simulink model "KUKA_Dynamics_internal_massonly"  (R2021b)
settings: Solver=ode4  StartTime=0.0  StopTime=0.01  FixedStep=0.01  RelTol=1e-3
InitFcn:
  | % ************** Initiate forces
  | % f0=[0;0;0;0;0;0];
  | % f0=[0;0;0;0;0;0;0];
  | %f_0=[0;0;0];
  | %f_m=[0;0];
  | %f_e=[0;0;0;0;0;0];
  | % ************** Initiate states
  | %q_m=[0;0];
  | %q_dot_m=[0;0];
  | %P=[0;0;0];
  | %V_I0=[0;0;0];
  | % ************** Load main
  | %run(Main.m)
values from neighbouring files (symbols this model uses):
  diag_M = diagonalize(M_frak0, M_frak)    [Create_Robot.m]    (also in Main.m; Main__iiwa7.m; diagonalize.m = zeros(6*(n+1),6*(n+1)); test_C_Main.m)
  f_e = [0;0;0;0;0;0]    [Create_Robot.m]    (also in Main.m = [0;0;0]; Main__iiwa7.m; test_C_Main.m)
  f_m = [0;0]    [Create_Robot.m]    (also in Main.m; Main__iiwa7.m; test_C_Main.m)
  q_dot_m = [0;0]    [Create_Robot.m]    (also in Main.m; Main__iiwa7.m; test_C_Main.m)
  q_m = [0;0]    [Create_Robot.m]    (also in Main.m = [0.2;0.4]; Main__iiwa7.m = [0.2;0.4]; test_C_Main.m = [1;0])
  X = [0 -x(3) x(2) ; x(3) 0 -x(1) ; -x(2) x(1) 0 ]    [skewsym.m]
  Xi_m_matrix = zeros(6*n,n)    [Create_Robot.m]    (also in Main.m; Main__iiwa7.m; test_C_Main.m)
undefined symbols (not defined in the file or in its folder): Xi_m, Y, Z
libraries: sm_lib x78, nesl_utility x29
(part 1 of 2)
settings Model: Creator=Bmmog  LastModifiedBy=Bmmog
settings SolverCC: AllowMultiTaskInputOutput=on

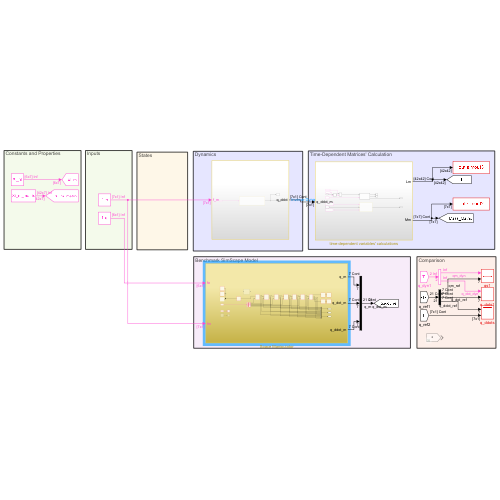
[thumbnail: Simulink's stored preview of the top-level diagram]
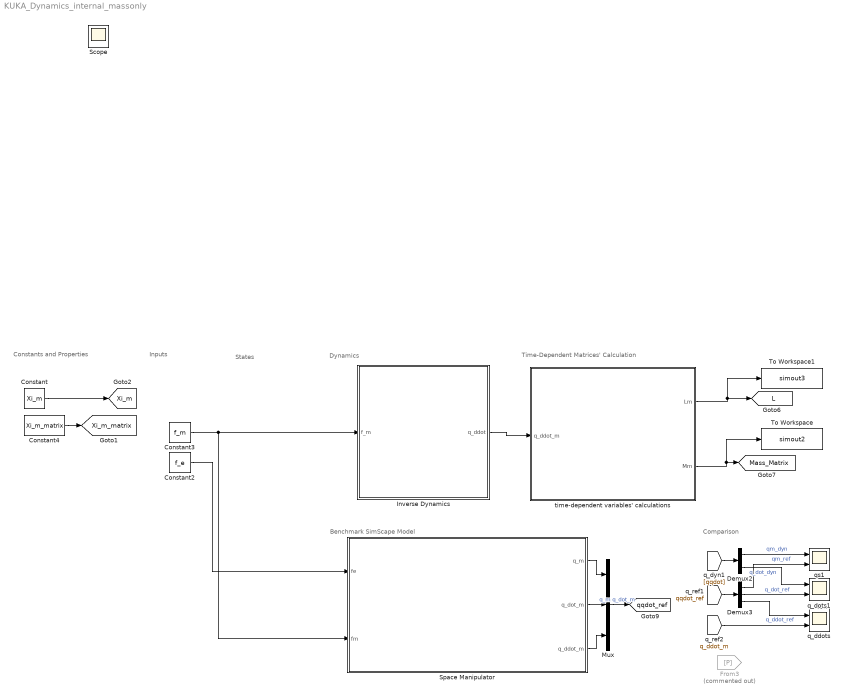
== system KUKA_Dynamics_internal_massonly ==
  note: Time-Dependent Matrices' Calculation
  note: States
  note: Inputs
  note: Dynamics
  note: Constants and Properties
  note: Benchmark SimScape Model
  note: Comparison
  Constant : Constant  Value=Xi_m  VectorParams1D=off
  Constant2 : Constant  Value=f_e  VectorParams1D=off
  Constant3 : Constant  Value=f_m  VectorParams1D=off
  Constant4 : Constant  Value=Xi_m_matrix  VectorParams1D=off
  Demux2 : Demux  Outputs=2
  Demux3 : Demux  Outputs=3
  From3 : From  Commented=on  GotoTag=P  TagVisibility=global
  Inverse Dynamics : Subsystem
  Mux : Mux  Inputs=3
  Space Manipulator : Subsystem
  To Workspace : ToWorkspace  VariableName=simout2  SaveFormat=Timeseries  SampleTime=-1
  To Workspace1 : ToWorkspace  VariableName=simout3  SaveFormat=Timeseries  SampleTime=-1
  q_ddots : Scope  NumInputPorts=2
  q_dots1 : Scope  NumInputPorts=2
  qs1 : Scope  NumInputPorts=2
  time-dependent variables' calculations : Subsystem
  Scope : Scope
  tag scope: L=global, Mass_Matrix=global, Xi_m=global, Xi_m_matrix=global, qqdot_ref=global
  wires:
  Constant/1 -> [Xi_m]
  Constant4/1 -> [Xi_m_matrix]
  time-dependent variables' calculations/2(Mm) -> To Workspace/1, [Mass_Matrix]
  time-dependent variables' calculations/1(Lm) -> To Workspace1/1, [L]
  Inverse Dynamics/1(q_ddot) -> time-dependent variables' calculations/1(q_ddot_m)
  Mux/1 -> [qqdot_ref]  "q_m q_dot_m"
  Constant2/1 -> Space Manipulator/1(fe)
  Space Manipulator/1(q_m) -> Mux/1
  Space Manipulator/2(q_dot_m) -> Mux/2
  Constant3/1 -> Space Manipulator/2(fm), Inverse Dynamics/1(f_m)
  Demux3/2 -> q_dots1/2  "q_dot_ref"
  [qqdot] -> Demux2/1
  Demux3/1 -> qs1/2  "qm_ref"
  Demux2/2 -> q_dots1/1  "q_dot_dyn"
  [qqdot_ref] -> Demux3/1
  Demux2/1 -> qs1/1  "qm_dyn"
  Space Manipulator/3(q_ddot_m) -> Mux/3
  Demux3/3 -> q_ddots/1  "q_ddot_ref"
  [q_ddot_m] -> q_ddots/2

== system KUKA_Dynamics_internal_massonly/Inverse Dynamics ==
  f_m : Inport
  Internal Dynamics : Subsystem
  q_ddot : Outport
  tag scope: q_ddot_m=global
  wires:
  f_m/1 -> Internal Dynamics/1(f_m)
  Internal Dynamics/1(q_ddot) -> [q_ddot_m], q_ddot/1  "q_ddot"

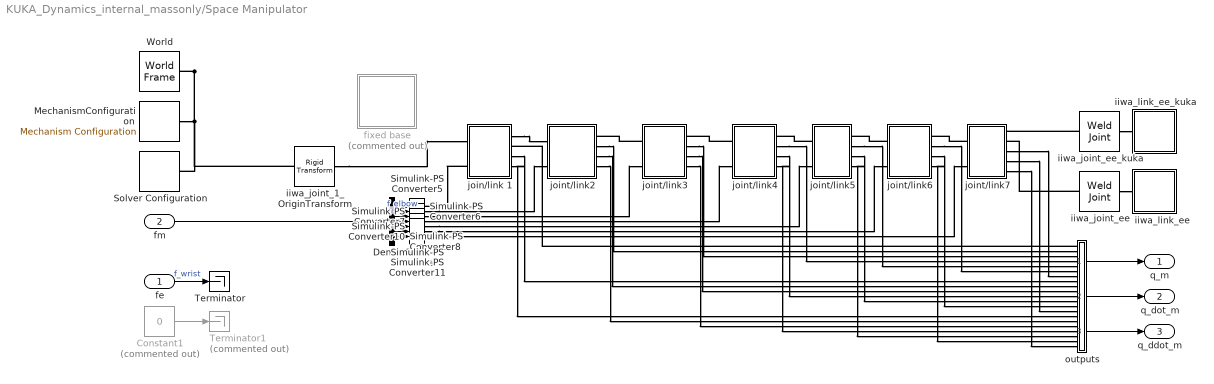
== system KUKA_Dynamics_internal_massonly/Space Manipulator ==
  fe : Inport
  fm : Inport  Port=2
  Constant1 : Constant  Commented=on  Value=0
  Demux2 : Demux  Outputs=7
  MechanismConfiguration : sm_lib/Utilities/Mechanism Configuration  UniformGravity=Constant  GravityVector=[0 0 0]  GravityUnits=m/s^2  LinearizationDelta=0.001  JointModeTransitionNonlinearIterations=2
  Simulink-PS Converter{5..11} (7 alike) : nesl_utility/Simulink-PS Converter  PhysicalDomain=network_engine_domain  SubClassName=ps_input  LeftPortType=input  RightPortType=output  PseudoPeriodic=off  Frequencies=[]  NoiseDistribution=none  NoiseParameters=[]  Unit=1  AffineConversion=off  FilteringAndDerivatives=provide  SimscapeFilterOrder=1  InputFilterTimeConstant=0.001  UdotUserProvided=0
      settings: SourceProductBaseCode=PW,SS
  Solver Configuration : nesl_utility/Solver Configuration  PhysicalDomain=network_engine_domain  SubClassName=solver  LeftPortType=input  RightPortType=generic  Tones=[]  Harmonics=[]  SimulateNoise=off  Profile=off  UseLocalSampling=off  EnableSwitchedLinearOptims=on  FrequencyDomain=off  UseCCode=off  RelTol=0.001  AbsTol=0.001  MinStep=1e-09  ToWorkspace=off  RevertToSquareIcSolve=off  NumHomotopyIterations=100  PhasorMode=off  PhasorModeNumHarmonics=1  DoDC=off  ResidualTolerance=1e-09  UseLocalSolver=off  LocalSolverChoice=NE_BACKWARD_EULER_ADVANCER  LocalSolverSampleTime=0.001  DoFixedCost=off  MaxNonlinIter=3  MaxModeIter=2  ComputeImpulses=off  ImpulseIterations=2  LinearAlgebra=auto  EquationFormulation=NE_TIME_EF  DelaysMemoryBudget=1024  AutomaticFiltering=on  FilteringTimeConstant=0.001  PartitionStorageMethod=AS_NEEDED  PartitionMemoryBudget=1024  PartitionMethod=ROBUST
      settings: SourceProductBaseCode=PW,SS
  Terminator : Terminator
  Terminator1 : Terminator  Commented=on
  World : sm_lib/Frames and Transforms/World Frame
  fixed base : Subsystem  Commented=on
  iiwa_joint_1_OriginTransform : sm_lib/Frames and Transforms/Rigid Transform  TranslationMethod=Cartesian  TranslationStandardOffset=0  TranslationLengthUnit=m  TranslationStandardAxis=+Z  TranslationCartesianOffset=[0, 0, 0]  TranslationROffset=0  TranslationROffsetUnits=m  TranslationZOffset=0  TranslationZOffsetUnits=m  TranslationThetaOffset=0  TranslationThetaOffsetUnits=deg  RotationMethod=RotationSequence  RotationAngleUnits=deg  RotationStandardAxis=+Z  RotationAngle=0.0  RotationArbitraryAxis=[0 0 1]  FollAlignAxisA=+X  BaseAlignAxisA=+Y  FollAlignAxisB=+Y  BaseAlignAxisB=+Z  RotationSequenceAxes=BaseAxes  RotationSequence=XYZ  RotationSequenceAngles=[0, 0, 0]  RotationSequenceAnglesUnits=rad  RotationMatrix=[1 0 0; 0 1 0; 0 0 1]
  iiwa_joint_ee : sm_lib/Joints/Weld Joint  JointMode=Normal  SenseConstraintForce=off  SenseConstraintForceX=off  SenseConstraintForceY=off  SenseConstraintForceZ=off  SenseConstraintTorque=off  SenseConstraintTorqueX=off  SenseConstraintTorqueY=off  SenseConstraintTorqueZ=off  SenseTotalForce=off  SenseTotalForceX=off  SenseTotalForceY=off  SenseTotalForceZ=off  SenseTotalTorque=off  SenseTotalTorqueX=off  SenseTotalTorqueY=off  SenseTotalTorqueZ=off  CompositeWrenchDir=FollowerOnBase  CompositeWrenchFrame=BaseFrame
  iiwa_joint_ee_kuka : sm_lib/Joints/Weld Joint  JointMode=Normal  SenseConstraintForce=off  SenseConstraintForceX=off  SenseConstraintForceY=off  SenseConstraintForceZ=off  SenseConstraintTorque=off  SenseConstraintTorqueX=off  SenseConstraintTorqueY=off  SenseConstraintTorqueZ=off  SenseTotalForce=off  SenseTotalForceX=off  SenseTotalForceY=off  SenseTotalForceZ=off  SenseTotalTorque=off  SenseTotalTorqueX=off  SenseTotalTorqueY=off  SenseTotalTorqueZ=off  CompositeWrenchDir=FollowerOnBase  CompositeWrenchFrame=BaseFrame
  iiwa_link_ee : Subsystem
  iiwa_link_ee_kuka : Subsystem
  join/link 1 : Subsystem
  joint/link2 : Subsystem
  joint/link3 : Subsystem
  joint/link4 : Subsystem
  joint/link5 : Subsystem
  joint/link6 : Subsystem
  joint/link7 : Subsystem
  outputs : Subsystem
  q_m : Outport
  q_dot_m : Outport  Port=2
  q_ddot_m : Outport  Port=3
  wires:
  fe/1 -> Terminator/1  "f_wrist"
  Demux2/7 -> Simulink-PS Converter11/1
  Demux2/1 -> Simulink-PS Converter5/1
  Demux2/5 -> Simulink-PS Converter9/1
  Demux2/2 -> Simulink-PS Converter6/1  "f_elbow"
  Constant1/1 -> Terminator1/1
  Demux2/4 -> Simulink-PS Converter8/1
  Demux2/6 -> Simulink-PS Converter10/1
  Demux2/3 -> Simulink-PS Converter7/1
  fm/1 -> Demux2/1
  outputs/1(q_m) -> q_m/1
  outputs/2(q_dot_m) -> q_dot_m/1
  outputs/3(q_ddot_m) -> q_ddot_m/1
  connections:
  World/RConn1 -- iiwa_joint_1_OriginTransform/LConn1 -- Solver Configuration/RConn1 -- MechanismConfiguration/RConn1
  joint/link7/RConn5 -- outputs/LConn21
  Simulink-PS Converter9/RConn1 -- joint/link5/LConn2
  Simulink-PS Converter7/RConn1 -- joint/link3/LConn2
  joint/link7/RConn4 -- outputs/LConn14
  joint/link3/RConn3 -- outputs/LConn10
  joint/link4/LConn1 -- joint/link3/RConn1
  join/link 1/RConn1 -- joint/link2/LConn1
  joint/link5/RConn4 -- outputs/LConn19
  outputs/LConn1 -- join/link 1/RConn2
  joint/link5/RConn2 -- outputs/LConn5
  joint/link6/RConn2 -- outputs/LConn6
  joint/link5/RConn3 -- outputs/LConn12
  joint/link7/LConn1 -- joint/link6/RConn1
  iiwa_joint_ee_kuka/LConn1 -- joint/link7/RConn1
  iiwa_joint_ee/RConn1 -- iiwa_link_ee/LConn1
  joint/link2/RConn2 -- outputs/LConn2
  joint/link2/RConn4 -- outputs/LConn16
  iiwa_joint_ee_kuka/RConn1 -- iiwa_link_ee_kuka/LConn1
  Simulink-PS Converter6/RConn1 -- joint/link2/LConn2
  joint/link4/RConn4 -- outputs/LConn18
  joint/link7/RConn3 -- outputs/LConn7
  Simulink-PS Converter8/RConn1 -- joint/link4/LConn2
  joint/link3/LConn1 -- joint/link2/RConn1
  iiwa_joint_ee/LConn1 -- joint/link7/RConn2
  join/link 1/RConn4 -- outputs/LConn15
  Simulink-PS Converter10/RConn1 -- joint/link6/LConn2
  joint/link3/RConn2 -- outputs/LConn3
  joint/link3/RConn4 -- outputs/LConn17
  joint/link6/RConn4 -- outputs/LConn20
  joint/link4/RConn2 -- outputs/LConn4
  joint/link6/LConn1 -- joint/link5/RConn1
  joint/link5/LConn1 -- joint/link4/RConn1
  join/link 1/RConn3 -- outputs/LConn8
  joint/link2/RConn3 -- outputs/LConn9
  joint/link6/RConn3 -- outputs/LConn13
  joint/link4/RConn3 -- outputs/LConn11
  Simulink-PS Converter11/RConn1 -- joint/link7/LConn2
  iiwa_joint_1_OriginTransform/RConn1 -- join/link 1/LConn1
  join/link 1/LConn2 -- Simulink-PS Converter5/RConn1

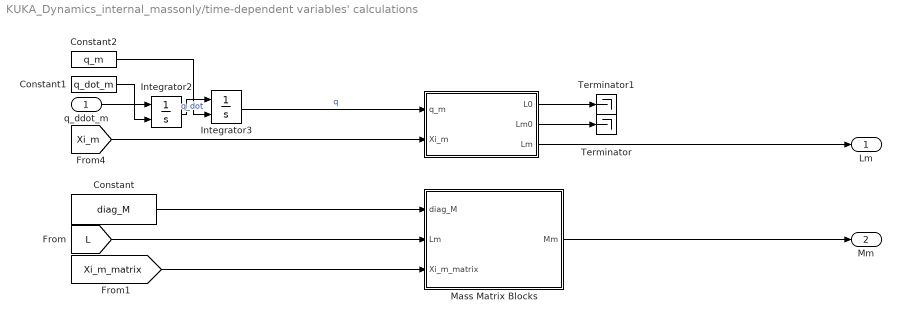
== system KUKA_Dynamics_internal_massonly/time-dependent variables' calculations ==
  q_ddot_m : Inport
  " " : MATLAB Function  TreatAsAtomicUnit=on
  Constant : Constant  Value=diag_M  VectorParams1D=off
  Constant1 : Constant  Value=q_dot_m  VectorParams1D=off
  Constant2 : Constant  Value=q_m  VectorParams1D=off
  Integrator2 : Integrator  InitialConditionSource=external  InitialCondition=q_dot_m
  Integrator3 : Integrator  InitialConditionSource=external
  Mass Matrix Blocks : Subsystem
  Terminator : Terminator
  Terminator1 : Terminator
  Lm : Outport
  Mm : Outport  Port=2
  wires:
  Mass Matrix Blocks/1(Mm) -> Mm/1
  Integrator2/1 -> Integrator3/1  "q_dot"
  q_ddot_m/1 -> Integrator2/1
  " "/1(L0) -> Terminator1/1
  " "/3(Lm) -> Lm/1
  " "/2(Lm0) -> Terminator/1
  Constant/1 -> Mass Matrix Blocks/1(diag_M)
  [L] -> Mass Matrix Blocks/2(Lm)
  [Xi_m_matrix] -> Mass Matrix Blocks/3(Xi_m_matrix)
  [Xi_m] -> " "/2(Xi_m)
  Integrator3/1 -> " "/1(q_m)  "q"
  Constant1/1 -> Integrator2/2
  Constant2/1 -> Integrator3/2

== system KUKA_Dynamics_internal_massonly/Inverse Dynamics/Internal Dynamics ==
  f_m : Inport
  Divide : Product  Inputs=/*  Multiplication=Matrix(*)
  To Workspace : ToWorkspace  VariableName=qddot  SaveFormat=Timeseries  SampleTime=-1
  q_ddot : Outport
  wires:
  f_m/1 -> Divide/2
  Divide/1 -> To Workspace/1, q_ddot/1
  [Mass_Matrix] -> Divide/1

== system KUKA_Dynamics_internal_massonly/Space Manipulator/fixed base ==
  iiwa_link_0 : Subsystem
  world_iiwa_joint : sm_lib/Joints/Weld Joint  JointMode=Normal  SenseConstraintForce=off  SenseConstraintForceX=off  SenseConstraintForceY=off  SenseConstraintForceZ=off  SenseConstraintTorque=off  SenseConstraintTorqueX=off  SenseConstraintTorqueY=off  SenseConstraintTorqueZ=off  SenseTotalForce=off  SenseTotalForceX=off  SenseTotalForceY=off  SenseTotalForceZ=off  SenseTotalTorque=off  SenseTotalTorqueX=off  SenseTotalTorqueY=off  SenseTotalTorqueZ=off  CompositeWrenchDir=FollowerOnBase  CompositeWrenchFrame=BaseFrame
  F1 : PMIOPort  Side=Right
  Conn2 : PMIOPort  Port=2  Side=Left
  connections:
  iiwa_link_0/LConn1 -- world_iiwa_joint/RConn1
  Conn2/RConn1 -- world_iiwa_joint/LConn1
  F1/RConn1 -- iiwa_link_0/RConn1

== system KUKA_Dynamics_internal_massonly/Space Manipulator/iiwa_link_ee ==
  ReferenceFrame : sm_lib/Frames and Transforms/Reference Frame
  F : PMIOPort  Side=Left
  connections:
  ReferenceFrame/RConn1 -- F/RConn1

== system KUKA_Dynamics_internal_massonly/Space Manipulator/iiwa_link_ee_kuka ==
  ReferenceFrame : sm_lib/Frames and Transforms/Reference Frame
  F : PMIOPort  Side=Left
  connections:
  ReferenceFrame/RConn1 -- F/RConn1

== system KUKA_Dynamics_internal_massonly/Space Manipulator/join//link 1 ==
  iiwa_joint_1 : sm_lib/Joints/Revolute Joint  JointMode=Normal  SenseConstraintForce=off  SenseConstraintForceX=off  SenseConstraintForceY=off  SenseConstraintForceZ=off  SenseConstraintTorque=off  SenseConstraintTorqueX=off  SenseConstraintTorqueY=off  SenseConstraintTorqueZ=off  SenseTotalForce=off  SenseTotalForceX=off  SenseTotalForceY=off  SenseTotalForceZ=off  SenseTotalTorque=off  SenseTotalTorqueX=off  SenseTotalTorqueY=off  SenseTotalTorqueZ=off  CompositeWrenchDir=FollowerOnBase  CompositeWrenchFrame=BaseFrame  EquilibriumPosition=0  EquilibriumPositionUnits=deg  SpringStiffness=0  SpringStiffnessUnits=N*m/deg  DampingCoefficient=0.5  DampingCoefficientUnits=kg*m^2/(rad*s)  TorqueActuationMode=InputTorque  MotionActuationMode=ComputedMotion  SensePosition=on  SenseVelocity=on  SenseAcceleration=on  SenseTorqueForce=off  SenseLowerLimitTorqueForce=off  SenseUpperLimitTorqueForce=off  LowerLimitSpecify=on  LowerLimitBound=-2.96705972839  LowerLimitBoundUnits=rad  LowerLimitStiffness=1e4  LowerLimitStiffnessUnits=N*m/deg  LowerLimitDamping=10  LowerLimitDampingUnits=N*m/(deg/s)  LowerLimitTransitionRegionWidth=0.1  LowerLimitTransitionRegionWidthUnits=deg  UpperLimitSpecify=on  UpperLimitBound=2.96705972839  UpperLimitBoundUnits=rad  UpperLimitStiffness=1e4  UpperLimitStiffnessUnits=N*m/deg  UpperLimitDamping=10  UpperLimitDampingUnits=N*m/(deg/s)  UpperLimitTransitionRegionWidth=0.1  UpperLimitTransitionRegionWidthUnits=deg  PositionTargetSpecify=on  PositionTargetPriority=High  PositionTargetValue=q_m(1)  PositionTargetValueUnits=rad  VelocityTargetSpecify=on  VelocityTargetPriority=High  VelocityTargetValue=0  VelocityTargetValueUnits=rad/s
  iiwa_link_1 : Subsystem
  b : PMIOPort  Side=Left
  f1 : PMIOPort  Port=2  Side=Left
  F1 : PMIOPort  Port=3  Side=Right
  q1 : PMIOPort  Port=4  Side=Right
  qd1 : PMIOPort  Port=5  Side=Right
  qdd1 : PMIOPort  Port=6  Side=Right
  connections:
  iiwa_joint_1/RConn1 -- iiwa_link_1/LConn1
  iiwa_joint_1/LConn1 -- b/RConn1
  iiwa_joint_1/RConn2 -- q1/RConn1
  f1/RConn1 -- iiwa_joint_1/LConn2
  iiwa_joint_1/RConn3 -- qd1/RConn1
  iiwa_joint_1/RConn4 -- qdd1/RConn1
  F1/RConn1 -- iiwa_link_1/RConn1

== system KUKA_Dynamics_internal_massonly/Space Manipulator/joint//link2 ==
  iiwa_joint_2 : sm_lib/Joints/Revolute Joint  JointMode=Normal  SenseConstraintForce=off  SenseConstraintForceX=off  SenseConstraintForceY=off  SenseConstraintForceZ=off  SenseConstraintTorque=off  SenseConstraintTorqueX=off  SenseConstraintTorqueY=off  SenseConstraintTorqueZ=off  SenseTotalForce=off  SenseTotalForceX=off  SenseTotalForceY=off  SenseTotalForceZ=off  SenseTotalTorque=off  SenseTotalTorqueX=off  SenseTotalTorqueY=off  SenseTotalTorqueZ=off  CompositeWrenchDir=FollowerOnBase  CompositeWrenchFrame=BaseFrame  EquilibriumPosition=0  EquilibriumPositionUnits=deg  SpringStiffness=0  SpringStiffnessUnits=N*m/deg  DampingCoefficient=0.5  DampingCoefficientUnits=kg*m^2/(rad*s)  TorqueActuationMode=InputTorque  MotionActuationMode=ComputedMotion  SensePosition=on  SenseVelocity=on  SenseAcceleration=on  SenseTorqueForce=off  SenseLowerLimitTorqueForce=off  SenseUpperLimitTorqueForce=off  LowerLimitSpecify=on  LowerLimitBound=-2.09439510239  LowerLimitBoundUnits=rad  LowerLimitStiffness=1e4  LowerLimitStiffnessUnits=N*m/deg  LowerLimitDamping=10  LowerLimitDampingUnits=N*m/(deg/s)  LowerLimitTransitionRegionWidth=0.1  LowerLimitTransitionRegionWidthUnits=deg  UpperLimitSpecify=on  UpperLimitBound=2.09439510239  UpperLimitBoundUnits=rad  UpperLimitStiffness=1e4  UpperLimitStiffnessUnits=N*m/deg  UpperLimitDamping=10  UpperLimitDampingUnits=N*m/(deg/s)  UpperLimitTransitionRegionWidth=0.1  UpperLimitTransitionRegionWidthUnits=deg  PositionTargetSpecify=on  PositionTargetPriority=High  PositionTargetValue=q_m(2)  PositionTargetValueUnits=rad  VelocityTargetSpecify=on  VelocityTargetPriority=High  VelocityTargetValue=0  VelocityTargetValueUnits=rad/s
  iiwa_link_2 : Subsystem
  b : PMIOPort  Side=Left
  F1 : PMIOPort  Port=2  Side=Right
  f2 : PMIOPort  Port=3  Side=Left
  q2 : PMIOPort  Port=4  Side=Right
  qd2 : PMIOPort  Port=5  Side=Right
  qdd2 : PMIOPort  Port=6  Side=Right
  connections:
  iiwa_joint_2/RConn3 -- qd2/RConn1
  iiwa_joint_2/RConn1 -- iiwa_link_2/LConn1
  F1/RConn1 -- iiwa_link_2/RConn1
  iiwa_joint_2/RConn4 -- qdd2/RConn1
  iiwa_joint_2/LConn1 -- b/RConn1
  f2/RConn1 -- iiwa_joint_2/LConn2
  iiwa_joint_2/RConn2 -- q2/RConn1

== system KUKA_Dynamics_internal_massonly/Space Manipulator/joint//link3 ==
  iiwa_joint_3 : sm_lib/Joints/Revolute Joint  JointMode=Normal  SenseConstraintForce=off  SenseConstraintForceX=off  SenseConstraintForceY=off  SenseConstraintForceZ=off  SenseConstraintTorque=off  SenseConstraintTorqueX=off  SenseConstraintTorqueY=off  SenseConstraintTorqueZ=off  SenseTotalForce=off  SenseTotalForceX=off  SenseTotalForceY=off  SenseTotalForceZ=off  SenseTotalTorque=off  SenseTotalTorqueX=off  SenseTotalTorqueY=off  SenseTotalTorqueZ=off  CompositeWrenchDir=FollowerOnBase  CompositeWrenchFrame=BaseFrame  EquilibriumPosition=0  EquilibriumPositionUnits=deg  SpringStiffness=0  SpringStiffnessUnits=N*m/deg  DampingCoefficient=0.5  DampingCoefficientUnits=kg*m^2/(rad*s)  TorqueActuationMode=InputTorque  MotionActuationMode=ComputedMotion  SensePosition=on  SenseVelocity=on  SenseAcceleration=on  SenseTorqueForce=off  SenseLowerLimitTorqueForce=off  SenseUpperLimitTorqueForce=off  LowerLimitSpecify=on  LowerLimitBound=-2.96705972839  LowerLimitBoundUnits=rad  LowerLimitStiffness=1e4  LowerLimitStiffnessUnits=N*m/deg  LowerLimitDamping=10  LowerLimitDampingUnits=N*m/(deg/s)  LowerLimitTransitionRegionWidth=0.1  LowerLimitTransitionRegionWidthUnits=deg  UpperLimitSpecify=on  UpperLimitBound=2.96705972839  UpperLimitBoundUnits=rad  UpperLimitStiffness=1e4  UpperLimitStiffnessUnits=N*m/deg  UpperLimitDamping=10  UpperLimitDampingUnits=N*m/(deg/s)  UpperLimitTransitionRegionWidth=0.1  UpperLimitTransitionRegionWidthUnits=deg  PositionTargetSpecify=on  PositionTargetPriority=High  PositionTargetValue=q_m(3)  PositionTargetValueUnits=rad  VelocityTargetSpecify=on  VelocityTargetPriority=High  VelocityTargetValue=0  VelocityTargetValueUnits=rad/s
  iiwa_link_3 : Subsystem
  b : PMIOPort  Side=Left
  F1 : PMIOPort  Port=2  Side=Right
  f3 : PMIOPort  Port=3  Side=Left
  q3 : PMIOPort  Port=4  Side=Right
  qd3 : PMIOPort  Port=5  Side=Right
  qdd3 : PMIOPort  Port=6  Side=Right
  connections:
  iiwa_joint_3/RConn1 -- iiwa_link_3/LConn1
  iiwa_joint_3/RConn4 -- qdd3/RConn1
  iiwa_joint_3/RConn3 -- qd3/RConn1
  iiwa_joint_3/RConn2 -- q3/RConn1
  F1/RConn1 -- iiwa_link_3/RConn1
  f3/RConn1 -- iiwa_joint_3/LConn2
  iiwa_joint_3/LConn1 -- b/RConn1

== system KUKA_Dynamics_internal_massonly/Space Manipulator/joint//link4 ==
  iiwa_joint_4 : sm_lib/Joints/Revolute Joint  JointMode=Normal  SenseConstraintForce=off  SenseConstraintForceX=off  SenseConstraintForceY=off  SenseConstraintForceZ=off  SenseConstraintTorque=off  SenseConstraintTorqueX=off  SenseConstraintTorqueY=off  SenseConstraintTorqueZ=off  SenseTotalForce=off  SenseTotalForceX=off  SenseTotalForceY=off  SenseTotalForceZ=off  SenseTotalTorque=off  SenseTotalTorqueX=off  SenseTotalTorqueY=off  SenseTotalTorqueZ=off  CompositeWrenchDir=FollowerOnBase  CompositeWrenchFrame=BaseFrame  EquilibriumPosition=0  EquilibriumPositionUnits=deg  SpringStiffness=0  SpringStiffnessUnits=N*m/deg  DampingCoefficient=0.5  DampingCoefficientUnits=kg*m^2/(rad*s)  TorqueActuationMode=InputTorque  MotionActuationMode=ComputedMotion  SensePosition=on  SenseVelocity=on  SenseAcceleration=on  SenseTorqueForce=off  SenseLowerLimitTorqueForce=off  SenseUpperLimitTorqueForce=off  LowerLimitSpecify=on  LowerLimitBound=-2.09439510239  LowerLimitBoundUnits=rad  LowerLimitStiffness=1e4  LowerLimitStiffnessUnits=N*m/deg  LowerLimitDamping=10  LowerLimitDampingUnits=N*m/(deg/s)  LowerLimitTransitionRegionWidth=0.1  LowerLimitTransitionRegionWidthUnits=deg  UpperLimitSpecify=on  UpperLimitBound=2.09439510239  UpperLimitBoundUnits=rad  UpperLimitStiffness=1e4  UpperLimitStiffnessUnits=N*m/deg  UpperLimitDamping=10  UpperLimitDampingUnits=N*m/(deg/s)  UpperLimitTransitionRegionWidth=0.1  UpperLimitTransitionRegionWidthUnits=deg  PositionTargetSpecify=on  PositionTargetPriority=High  PositionTargetValue=q_m(4)  PositionTargetValueUnits=rad  VelocityTargetSpecify=on  VelocityTargetPriority=High  VelocityTargetValue=0  VelocityTargetValueUnits=rad/s
  iiwa_link_4 : Subsystem
  b : PMIOPort  Side=Left
  F1 : PMIOPort  Port=2  Side=Right
  f4 : PMIOPort  Port=3  Side=Left
  q4 : PMIOPort  Port=4  Side=Right
  qd4 : PMIOPort  Port=5  Side=Right
  qd5 : PMIOPort  Port=6  Side=Right
  connections:
  iiwa_joint_4/RConn1 -- iiwa_link_4/LConn1
  iiwa_joint_4/RConn3 -- qd4/RConn1
  f4/RConn1 -- iiwa_joint_4/LConn2
  F1/RConn1 -- iiwa_link_4/RConn1
  iiwa_joint_4/RConn2 -- q4/RConn1
  iiwa_joint_4/LConn1 -- b/RConn1
  iiwa_joint_4/RConn4 -- qd5/RConn1

== system KUKA_Dynamics_internal_massonly/Space Manipulator/joint//link5 ==
  iiwa_joint_5 : sm_lib/Joints/Revolute Joint  JointMode=Normal  SenseConstraintForce=off  SenseConstraintForceX=off  SenseConstraintForceY=off  SenseConstraintForceZ=off  SenseConstraintTorque=off  SenseConstraintTorqueX=off  SenseConstraintTorqueY=off  SenseConstraintTorqueZ=off  SenseTotalForce=off  SenseTotalForceX=off  SenseTotalForceY=off  SenseTotalForceZ=off  SenseTotalTorque=off  SenseTotalTorqueX=off  SenseTotalTorqueY=off  SenseTotalTorqueZ=off  CompositeWrenchDir=FollowerOnBase  CompositeWrenchFrame=BaseFrame  EquilibriumPosition=0  EquilibriumPositionUnits=deg  SpringStiffness=0  SpringStiffnessUnits=N*m/deg  DampingCoefficient=0.5  DampingCoefficientUnits=kg*m^2/(rad*s)  TorqueActuationMode=InputTorque  MotionActuationMode=ComputedMotion  SensePosition=on  SenseVelocity=on  SenseAcceleration=on  SenseTorqueForce=off  SenseLowerLimitTorqueForce=off  SenseUpperLimitTorqueForce=off  LowerLimitSpecify=on  LowerLimitBound=-2.96705972839  LowerLimitBoundUnits=rad  LowerLimitStiffness=1e4  LowerLimitStiffnessUnits=N*m/deg  LowerLimitDamping=10  LowerLimitDampingUnits=N*m/(deg/s)  LowerLimitTransitionRegionWidth=0.1  LowerLimitTransitionRegionWidthUnits=deg  UpperLimitSpecify=on  UpperLimitBound=2.96705972839  UpperLimitBoundUnits=rad  UpperLimitStiffness=1e4  UpperLimitStiffnessUnits=N*m/deg  UpperLimitDamping=10  UpperLimitDampingUnits=N*m/(deg/s)  UpperLimitTransitionRegionWidth=0.1  UpperLimitTransitionRegionWidthUnits=deg  PositionTargetSpecify=on  PositionTargetPriority=High  PositionTargetValue=q_m(5)  PositionTargetValueUnits=rad  VelocityTargetSpecify=on  VelocityTargetPriority=High  VelocityTargetValue=0  VelocityTargetValueUnits=rad/s
  iiwa_link_5 : Subsystem
  b : PMIOPort  Side=Left
  F1 : PMIOPort  Port=2  Side=Right
  f5 : PMIOPort  Port=3  Side=Left
  q5 : PMIOPort  Port=4  Side=Right
  qd5 : PMIOPort  Port=5  Side=Right
  qdd5 : PMIOPort  Port=6  Side=Right
  connections:
  iiwa_joint_5/LConn1 -- b/RConn1
  iiwa_joint_5/RConn2 -- q5/RConn1
  iiwa_joint_5/RConn4 -- qdd5/RConn1
  iiwa_joint_5/RConn1 -- iiwa_link_5/LConn1
  iiwa_joint_5/RConn3 -- qd5/RConn1
  f5/RConn1 -- iiwa_joint_5/LConn2
  F1/RConn1 -- iiwa_link_5/RConn1

== system KUKA_Dynamics_internal_massonly/Space Manipulator/joint//link6 ==
  iiwa_joint_6 : sm_lib/Joints/Revolute Joint  JointMode=Normal  SenseConstraintForce=off  SenseConstraintForceX=off  SenseConstraintForceY=off  SenseConstraintForceZ=off  SenseConstraintTorque=off  SenseConstraintTorqueX=off  SenseConstraintTorqueY=off  SenseConstraintTorqueZ=off  SenseTotalForce=off  SenseTotalForceX=off  SenseTotalForceY=off  SenseTotalForceZ=off  SenseTotalTorque=off  SenseTotalTorqueX=off  SenseTotalTorqueY=off  SenseTotalTorqueZ=off  CompositeWrenchDir=FollowerOnBase  CompositeWrenchFrame=BaseFrame  EquilibriumPosition=0  EquilibriumPositionUnits=deg  SpringStiffness=0  SpringStiffnessUnits=N*m/deg  DampingCoefficient=0.5  DampingCoefficientUnits=kg*m^2/(rad*s)  TorqueActuationMode=InputTorque  MotionActuationMode=ComputedMotion  SensePosition=on  SenseVelocity=on  SenseAcceleration=on  SenseTorqueForce=off  SenseLowerLimitTorqueForce=off  SenseUpperLimitTorqueForce=off  LowerLimitSpecify=on  LowerLimitBound=-2.09439510239  LowerLimitBoundUnits=rad  LowerLimitStiffness=1e4  LowerLimitStiffnessUnits=N*m/deg  LowerLimitDamping=10  LowerLimitDampingUnits=N*m/(deg/s)  LowerLimitTransitionRegionWidth=0.1  LowerLimitTransitionRegionWidthUnits=deg  UpperLimitSpecify=on  UpperLimitBound=2.09439510239  UpperLimitBoundUnits=rad  UpperLimitStiffness=1e4  UpperLimitStiffnessUnits=N*m/deg  UpperLimitDamping=10  UpperLimitDampingUnits=N*m/(deg/s)  UpperLimitTransitionRegionWidth=0.1  UpperLimitTransitionRegionWidthUnits=deg  PositionTargetSpecify=on  PositionTargetPriority=High  PositionTargetValue=q_m(6)  PositionTargetValueUnits=rad  VelocityTargetSpecify=on  VelocityTargetPriority=High  VelocityTargetValue=0  VelocityTargetValueUnits=rad/s
  iiwa_link_6 : Subsystem
  b : PMIOPort  Side=Left
  F1 : PMIOPort  Port=2  Side=Right
  q6 : PMIOPort  Port=3  Side=Right
  f6 : PMIOPort  Port=4  Side=Left
  qd6 : PMIOPort  Port=5  Side=Right
  qdd6 : PMIOPort  Port=6  Side=Right
  connections:
  iiwa_joint_6/RConn1 -- iiwa_link_6/LConn1
  iiwa_joint_6/LConn1 -- b/RConn1
  F1/RConn1 -- iiwa_link_6/RConn1
  f6/RConn1 -- iiwa_joint_6/LConn2
  iiwa_joint_6/RConn4 -- qdd6/RConn1
  iiwa_joint_6/RConn3 -- qd6/RConn1
  iiwa_joint_6/RConn2 -- q6/RConn1

== system KUKA_Dynamics_internal_massonly/Space Manipulator/joint//link7 ==
  iiwa_joint_7 : sm_lib/Joints/Revolute Joint  JointMode=Normal  SenseConstraintForce=off  SenseConstraintForceX=off  SenseConstraintForceY=off  SenseConstraintForceZ=off  SenseConstraintTorque=off  SenseConstraintTorqueX=off  SenseConstraintTorqueY=off  SenseConstraintTorqueZ=off  SenseTotalForce=off  SenseTotalForceX=off  SenseTotalForceY=off  SenseTotalForceZ=off  SenseTotalTorque=off  SenseTotalTorqueX=off  SenseTotalTorqueY=off  SenseTotalTorqueZ=off  CompositeWrenchDir=FollowerOnBase  CompositeWrenchFrame=BaseFrame  EquilibriumPosition=0  EquilibriumPositionUnits=deg  SpringStiffness=0  SpringStiffnessUnits=N*m/deg  DampingCoefficient=0.5  DampingCoefficientUnits=kg*m^2/(rad*s)  TorqueActuationMode=InputTorque  MotionActuationMode=ComputedMotion  SensePosition=on  SenseVelocity=on  SenseAcceleration=on  SenseTorqueForce=off  SenseLowerLimitTorqueForce=off  SenseUpperLimitTorqueForce=off  LowerLimitSpecify=on  LowerLimitBound=-3.05432619099  LowerLimitBoundUnits=rad  LowerLimitStiffness=1e4  LowerLimitStiffnessUnits=N*m/deg  LowerLimitDamping=10  LowerLimitDampingUnits=N*m/(deg/s)  LowerLimitTransitionRegionWidth=0.1  LowerLimitTransitionRegionWidthUnits=deg  UpperLimitSpecify=on  UpperLimitBound=3.05432619099  UpperLimitBoundUnits=rad  UpperLimitStiffness=1e4  UpperLimitStiffnessUnits=N*m/deg  UpperLimitDamping=10  UpperLimitDampingUnits=N*m/(deg/s)  UpperLimitTransitionRegionWidth=0.1  UpperLimitTransitionRegionWidthUnits=deg  PositionTargetSpecify=on  PositionTargetPriority=High  PositionTargetValue=q_m(7)  PositionTargetValueUnits=rad  VelocityTargetSpecify=on  VelocityTargetPriority=High  VelocityTargetValue=0  VelocityTargetValueUnits=rad/s
  iiwa_link_7 : Subsystem
  F2 : PMIOPort  Side=Right
  b : PMIOPort  Port=2  Side=Left
  F1 : PMIOPort  Port=3  Side=Right
  q7 : PMIOPort  Port=4  Side=Right
  f7 : PMIOPort  Port=5  Side=Left
  qd7 : PMIOPort  Port=6  Side=Right
  qdd7 : PMIOPort  Port=7  Side=Right
  connections:
  iiwa_joint_7/RConn1 -- iiwa_link_7/LConn1
  iiwa_joint_7/RConn4 -- qdd7/RConn1
  iiwa_joint_7/RConn2 -- q7/RConn1
  iiwa_joint_7/RConn3 -- qd7/RConn1
  f7/RConn1 -- iiwa_joint_7/LConn2
  F1/RConn1 -- iiwa_link_7/RConn2
  F2/RConn1 -- iiwa_link_7/RConn1
  iiwa_joint_7/LConn1 -- b/RConn1

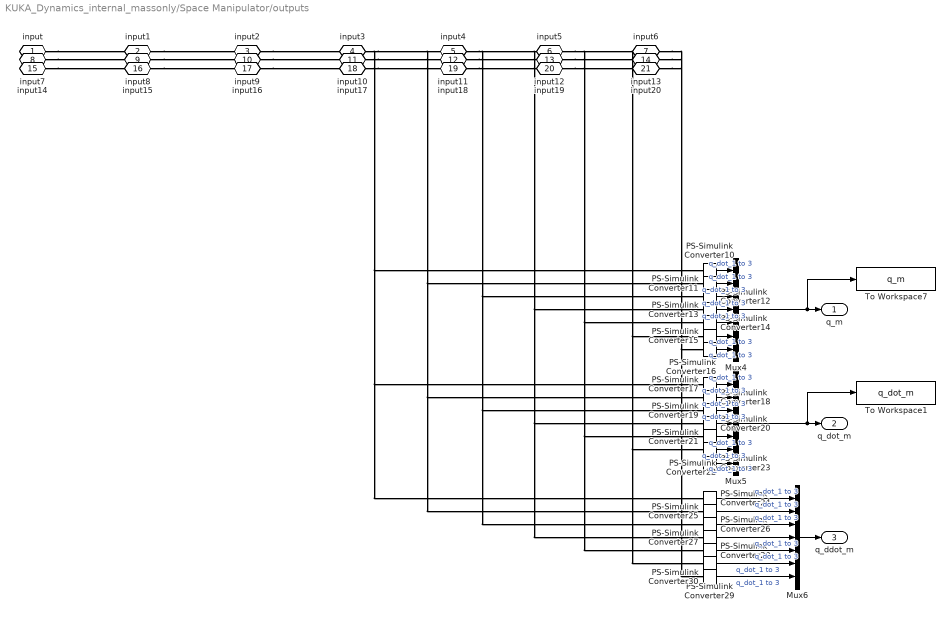
== system KUKA_Dynamics_internal_massonly/Space Manipulator/outputs ==
  Mux4 : Mux  Inputs=7
  Mux5 : Mux  Inputs=7
  Mux6 : Mux  Inputs=7
  PS-Simulink Converter{10..30} (21 alike) : nesl_utility/PS-Simulink Converter  PhysicalDomain=network_engine_domain  SubClassName=ps_output  LeftPortType=input  RightPortType=output  PseudoPeriodic=off  Frequencies=[]  Unit=inherit  AffineConversion=off
      settings: SourceProductBaseCode=PW,SS
  To Workspace1 : ToWorkspace  VariableName=q_dot_m  SampleTime=-1
  To Workspace7 : ToWorkspace  VariableName=q_m  SampleTime=-1
  input : PMIOPort  Side=Left
  input1 : PMIOPort  Port=2  Side=Left
  input2 : PMIOPort  Port=3  Side=Left
  input3 : PMIOPort  Port=4  Side=Left
  input4 : PMIOPort  Port=5  Side=Left
  input5 : PMIOPort  Port=6  Side=Left
  input6 : PMIOPort  Port=7  Side=Left
  input7 : PMIOPort  Port=8  Side=Left
  input8 : PMIOPort  Port=9  Side=Left
  input9 : PMIOPort  Port=10  Side=Left
  input10 : PMIOPort  Port=11  Side=Left
  input11 : PMIOPort  Port=12  Side=Left
  input12 : PMIOPort  Port=13  Side=Left
  input13 : PMIOPort  Port=14  Side=Left
  input14 : PMIOPort  Port=15  Side=Left
  input15 : PMIOPort  Port=16  Side=Left
  input16 : PMIOPort  Port=17  Side=Left
  input17 : PMIOPort  Port=18  Side=Left
  input18 : PMIOPort  Port=19  Side=Left
  input19 : PMIOPort  Port=20  Side=Left
  input20 : PMIOPort  Port=21  Side=Left
  q_m : Outport
  q_dot_m : Outport  Port=2
  q_ddot_m : Outport  Port=3
  wires:
  PS-Simulink Converter21/1 -> Mux5/5  "q_dot_1 to 3"
  PS-Simulink Converter12/1 -> Mux4/3  "q_dot_1 to 3"
  PS-Simulink Converter29/1 -> Mux6/6  "q_dot_1 to 3"
  PS-Simulink Converter14/1 -> Mux4/5  "q_dot_1 to 3"
  PS-Simulink Converter26/1 -> Mux6/3  "q_dot_1 to 3"
  PS-Simulink Converter17/1 -> Mux5/1  "q_dot_1 to 3"
  PS-Simulink Converter11/1 -> Mux4/2  "q_dot_1 to 3"
  PS-Simulink Converter25/1 -> Mux6/2  "q_dot_1 to 3"
  PS-Simulink Converter24/1 -> Mux6/1  "q_dot_1 to 3"
  PS-Simulink Converter10/1 -> Mux4/1  "q_dot_1 to 3"
  PS-Simulink Converter27/1 -> Mux6/4  "q_dot_1 to 3"
  PS-Simulink Converter28/1 -> Mux6/5  "q_dot_1 to 3"
  PS-Simulink Converter15/1 -> Mux4/6  "q_dot_1 to 3"
  PS-Simulink Converter16/1 -> Mux4/7  "q_dot_1 to 3"
  PS-Simulink Converter18/1 -> Mux5/2  "q_dot_1 to 3"
  PS-Simulink Converter30/1 -> Mux6/7  "q_dot_1 to 3"
  PS-Simulink Converter13/1 -> Mux4/4  "q_dot_1 to 3"
  PS-Simulink Converter22/1 -> Mux5/6  "q_dot_1 to 3"
  PS-Simulink Converter23/1 -> Mux5/7  "q_dot_1 to 3"
  PS-Simulink Converter20/1 -> Mux5/4  "q_dot_1 to 3"
  PS-Simulink Converter19/1 -> Mux5/3  "q_dot_1 to 3"
  Mux5/1 -> To Workspace1/1, q_dot_m/1
  Mux6/1 -> q_ddot_m/1
  Mux4/1 -> To Workspace7/1, q_m/1
  connections:
  input7/RConn1 -- PS-Simulink Converter17/LConn1
  input11/RConn1 -- PS-Simulink Converter21/LConn1
  input20/RConn1 -- PS-Simulink Converter30/LConn1
  input16/RConn1 -- PS-Simulink Converter26/LConn1
  input2/RConn1 -- PS-Simulink Converter12/LConn1
  input10/RConn1 -- PS-Simulink Converter20/LConn1
  input17/RConn1 -- PS-Simulink Converter27/LConn1
  input18/RConn1 -- PS-Simulink Converter28/LConn1
  input/RConn1 -- PS-Simulink Converter10/LConn1
  input19/RConn1 -- PS-Simulink Converter29/LConn1
  input5/RConn1 -- PS-Simulink Converter15/LConn1
  input14/RConn1 -- PS-Simulink Converter24/LConn1
  input6/RConn1 -- PS-Simulink Converter16/LConn1
  input9/RConn1 -- PS-Simulink Converter19/LConn1
  input8/RConn1 -- PS-Simulink Converter18/LConn1
  input15/RConn1 -- PS-Simulink Converter25/LConn1
  input12/RConn1 -- PS-Simulink Converter22/LConn1
  input13/RConn1 -- PS-Simulink Converter23/LConn1
  input1/RConn1 -- PS-Simulink Converter11/LConn1
  input4/RConn1 -- PS-Simulink Converter14/LConn1
  input3/RConn1 -- PS-Simulink Converter13/LConn1

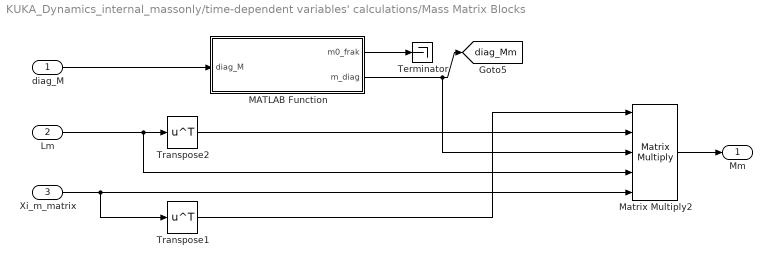
== system KUKA_Dynamics_internal_massonly/time-dependent variables' calculations/Mass Matrix Blocks ==
  diag_M : Inport
  Lm : Inport  Port=2
  Xi_m_matrix : Inport  Port=3
  MATLAB Function : MATLAB Function  TreatAsAtomicUnit=on
  Matrix Multiply2 : Product  Inputs=5  Multiplication=Matrix(*)
  Terminator : Terminator
  Transpose1 : Math  Operator=transpose  SaturateOnIntegerOverflow=on
  Transpose2 : Math  Operator=transpose  SaturateOnIntegerOverflow=on
  Mm : Outport
  tag scope: diag_Mm=global
  wires:
  Matrix Multiply2/1 -> Mm/1
  Xi_m_matrix/1 -> Transpose1/1, Matrix Multiply2/5
  diag_M/1 -> MATLAB Function/1(diag_M)
  Lm/1 -> Matrix Multiply2/4, Transpose2/1
  Transpose1/1 -> Matrix Multiply2/1
  Transpose2/1 -> Matrix Multiply2/2
  MATLAB Function/1(m0_frak) -> Terminator/1
  MATLAB Function/2(m_diag) -> [diag_Mm], Matrix Multiply2/3

== system KUKA_Dynamics_internal_massonly/Space Manipulator/fixed base/iiwa_link_0 ==
  Inertia : sm_lib/Body Elements/Inertia  InertiaType=Custom  Mass=5  MassUnits=kg  CenterOfMass=[0, 0, 0]  CenterOfMassUnits=m  MomentsOfInertia=[0.05, 0.06, 0.03]  MomentsOfInertiaUnits=kg*m^2  ProductsOfInertia=[0, 0, 0]  ProductsOfInertiaUnits=kg*m^2  GraphicType=None  MarkerShape=Inertia  MarkerSize=20  GraphicVisPropType=SimpleVisualProperties  GraphicDiffuseColor=[0.5 0.5 0.5]  GraphicSpecularColor=[0.5 0.5 0.5 1.0]  GraphicAmbientColor=[0.15 0.15 0.15 1.0]  GraphicEmissiveColor=[0.0 0.0 0.0 1.0]  GraphicShininess=75  GraphicOpacity=1.0
  InertiaOriginTransform : sm_lib/Frames and Transforms/Rigid Transform  TranslationMethod=Cartesian  TranslationStandardOffset=0  TranslationLengthUnit=m  TranslationStandardAxis=+Z  TranslationCartesianOffset=[-0.1, 0, 0.07000000000000001]  TranslationROffset=0  TranslationROffsetUnits=m  TranslationZOffset=0  TranslationZOffsetUnits=m  TranslationThetaOffset=0  TranslationThetaOffsetUnits=deg  RotationMethod=RotationSequence  RotationAngleUnits=deg  RotationStandardAxis=+Z  RotationAngle=0.0  RotationArbitraryAxis=[0 0 1]  FollAlignAxisA=+X  BaseAlignAxisA=+Y  FollAlignAxisB=+Y  BaseAlignAxisB=+Z  RotationSequenceAxes=BaseAxes  RotationSequence=XYZ  RotationSequenceAngles=[0, 0, 0]  RotationSequenceAnglesUnits=rad  RotationMatrix=[1 0 0; 0 1 0; 0 0 1]
  ReferenceFrame : sm_lib/Frames and Transforms/Reference Frame
  Visual : sm_lib/Body Elements/File Solid  ExtGeomFileName=iiwa_description/meshes/iiwa7/visual/link_0.stl  UnitType=Custom  ExtGeomFileUnits=m  StepReaderType=HEX  ExportConvexHullGeometry=off  InertiaType=Custom  Mass=0  MassUnits=kg  CenterOfMass=[0, 0, 0]  CenterOfMassUnits=m  MomentsOfInertia=[0, 0, 0]  MomentsOfInertiaUnits=kg*m^2  ProductsOfInertia=[0, 0, 0]  ProductsOfInertiaUnits=kg*m^2  BasedOnType=DensityFromFile  Density=1000  DensityUnits=kg/m^3  DoExposeReferenceFrame=on  SerializedFrames=<Frames/>  GraphicType=FromGeometry  MarkerShape=Sphere  MarkerSize=10  GraphicVisPropType=SimpleVisualProperties  GraphicDiffuseColor=[0.4, 0.4, 0.4]  GraphicSpecularColor=[0.5 0.5 0.5 1.0]  GraphicAmbientColor=[0.15 0.15 0.15 1.0]  GraphicEmissiveColor=[0.0 0.0 0.0 1.0]  GraphicShininess=75  GraphicOpacity=1
  VisualOriginTransform : sm_lib/Frames and Transforms/Rigid Transform  TranslationMethod=Cartesian  TranslationStandardOffset=0  TranslationLengthUnit=m  TranslationStandardAxis=+Z  TranslationCartesianOffset=[0, 0, 0]  TranslationROffset=0  TranslationROffsetUnits=m  TranslationZOffset=0  TranslationZOffsetUnits=m  TranslationThetaOffset=0  TranslationThetaOffsetUnits=deg  RotationMethod=RotationSequence  RotationAngleUnits=deg  RotationStandardAxis=+Z  RotationAngle=0.0  RotationArbitraryAxis=[0 0 1]  FollAlignAxisA=+X  BaseAlignAxisA=+Y  FollAlignAxisB=+Y  BaseAlignAxisB=+Z  RotationSequenceAxes=BaseAxes  RotationSequence=XYZ  RotationSequenceAngles=[0, 0, 0]  RotationSequenceAnglesUnits=rad  RotationMatrix=[1 0 0; 0 1 0; 0 0 1]
  iiwa_joint_1_AxisTransform : sm_lib/Frames and Transforms/Rigid Transform  TranslationMethod=Cartesian  TranslationStandardOffset=0  TranslationLengthUnit=m  TranslationStandardAxis=+Z  TranslationCartesianOffset=[0, 0, 0]  TranslationROffset=0  TranslationROffsetUnits=m  TranslationZOffset=0  TranslationZOffsetUnits=m  TranslationThetaOffset=0  TranslationThetaOffsetUnits=deg  RotationMethod=ArbitraryAxis  RotationAngleUnits=rad  RotationStandardAxis=+Z  RotationAngle=0  RotationArbitraryAxis=[1, 0, 0]  FollAlignAxisA=+X  BaseAlignAxisA=+Y  FollAlignAxisB=+Y  BaseAlignAxisB=+Z  RotationSequenceAxes=FollowerAxes  RotationSequence=XYX  RotationSequenceAngles=[0 0 0]  RotationSequenceAnglesUnits=deg  RotationMatrix=[1 0 0; 0 1 0; 0 0 1]
  iiwa_joint_1_OriginTransform : sm_lib/Frames and Transforms/Rigid Transform  TranslationMethod=Cartesian  TranslationStandardOffset=0  TranslationLengthUnit=m  TranslationStandardAxis=+Z  TranslationCartesianOffset=[0, 0, 0.02]  TranslationROffset=0  TranslationROffsetUnits=m  TranslationZOffset=0  TranslationZOffsetUnits=m  TranslationThetaOffset=0  TranslationThetaOffsetUnits=deg  RotationMethod=RotationSequence  RotationAngleUnits=deg  RotationStandardAxis=+Z  RotationAngle=0.0  RotationArbitraryAxis=[0 0 1]  FollAlignAxisA=+X  BaseAlignAxisA=+Y  FollAlignAxisB=+Y  BaseAlignAxisB=+Z  RotationSequenceAxes=BaseAxes  RotationSequence=XYZ  RotationSequenceAngles=[0, 0, 0]  RotationSequenceAnglesUnits=rad  RotationMatrix=[1 0 0; 0 1 0; 0 0 1]
  F : PMIOPort  Side=Left
  F1 : PMIOPort  Port=2  Side=Right
  connections:
  Inertia/RConn1 -- InertiaOriginTransform/RConn1
  InertiaOriginTransform/LConn1 -- ReferenceFrame/RConn1 -- F/RConn1 -- VisualOriginTransform/LConn1 -- iiwa_joint_1_OriginTransform/LConn1
  Visual/RConn1 -- VisualOriginTransform/RConn1
  iiwa_joint_1_AxisTransform/RConn1 -- F1/RConn1
  iiwa_joint_1_AxisTransform/LConn1 -- iiwa_joint_1_OriginTransform/RConn1

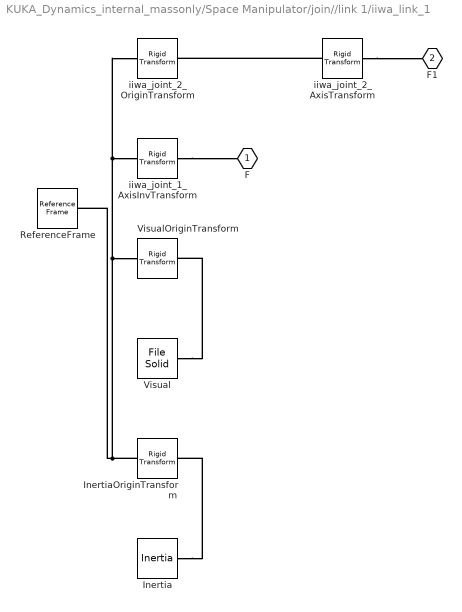
== system KUKA_Dynamics_internal_massonly/Space Manipulator/join//link 1/iiwa_link_1 ==
  Inertia : sm_lib/Body Elements/Inertia  InertiaType=Custom  Mass=3.4525  MassUnits=kg  CenterOfMass=[0, 0, 0]  CenterOfMassUnits=m  MomentsOfInertia=[0.02183, 0.007703, 0.02083]  MomentsOfInertiaUnits=kg*m^2  ProductsOfInertia=[-0.003887, 0, 0]  ProductsOfInertiaUnits=kg*m^2  GraphicType=None  MarkerShape=Inertia  MarkerSize=20  GraphicVisPropType=SimpleVisualProperties  GraphicDiffuseColor=[0.5 0.5 0.5]  GraphicSpecularColor=[0.5 0.5 0.5 1.0]  GraphicAmbientColor=[0.15 0.15 0.15 1.0]  GraphicEmissiveColor=[0.0 0.0 0.0 1.0]  GraphicShininess=75  GraphicOpacity=1.0
  InertiaOriginTransform : sm_lib/Frames and Transforms/Rigid Transform  TranslationMethod=Cartesian  TranslationStandardOffset=0  TranslationLengthUnit=m  TranslationStandardAxis=+Z  TranslationCartesianOffset=[0, -0.03, 0.12]  TranslationROffset=0  TranslationROffsetUnits=m  TranslationZOffset=0  TranslationZOffsetUnits=m  TranslationThetaOffset=0  TranslationThetaOffsetUnits=deg  RotationMethod=RotationSequence  RotationAngleUnits=deg  RotationStandardAxis=+Z  RotationAngle=0.0  RotationArbitraryAxis=[0 0 1]  FollAlignAxisA=+X  BaseAlignAxisA=+Y  FollAlignAxisB=+Y  BaseAlignAxisB=+Z  RotationSequenceAxes=BaseAxes  RotationSequence=XYZ  RotationSequenceAngles=[0, 0, 0]  RotationSequenceAnglesUnits=rad  RotationMatrix=[1 0 0; 0 1 0; 0 0 1]
  ReferenceFrame : sm_lib/Frames and Transforms/Reference Frame
  Visual : sm_lib/Body Elements/File Solid  ExtGeomFileName=iiwa_description/meshes/iiwa7/visual/link_1.stl  UnitType=Custom  ExtGeomFileUnits=m  StepReaderType=HEX  ExportConvexHullGeometry=off  InertiaType=Custom  Mass=0  MassUnits=kg  CenterOfMass=[0, 0, 0]  CenterOfMassUnits=m  MomentsOfInertia=[0, 0, 0]  MomentsOfInertiaUnits=kg*m^2  ProductsOfInertia=[0, 0, 0]  ProductsOfInertiaUnits=kg*m^2  BasedOnType=DensityFromFile  Density=1000  DensityUnits=kg/m^3  DoExposeReferenceFrame=on  SerializedFrames=<Frames/>  GraphicType=FromGeometry  MarkerShape=Sphere  MarkerSize=10  GraphicVisPropType=SimpleVisualProperties  GraphicDiffuseColor=[1, 0.423529411765, 0.0392156862745]  GraphicSpecularColor=[0.5 0.5 0.5 1.0]  GraphicAmbientColor=[0.15 0.15 0.15 1.0]  GraphicEmissiveColor=[0.0 0.0 0.0 1.0]  GraphicShininess=75  GraphicOpacity=1
  VisualOriginTransform : sm_lib/Frames and Transforms/Rigid Transform  TranslationMethod=Cartesian  TranslationStandardOffset=0  TranslationLengthUnit=m  TranslationStandardAxis=+Z  TranslationCartesianOffset=[0, 0, 0]  TranslationROffset=0  TranslationROffsetUnits=m  TranslationZOffset=0  TranslationZOffsetUnits=m  TranslationThetaOffset=0  TranslationThetaOffsetUnits=deg  RotationMethod=RotationSequence  RotationAngleUnits=deg  RotationStandardAxis=+Z  RotationAngle=0.0  RotationArbitraryAxis=[0 0 1]  FollAlignAxisA=+X  BaseAlignAxisA=+Y  FollAlignAxisB=+Y  BaseAlignAxisB=+Z  RotationSequenceAxes=BaseAxes  RotationSequence=XYZ  RotationSequenceAngles=[0, 0, 0]  RotationSequenceAnglesUnits=rad  RotationMatrix=[1 0 0; 0 1 0; 0 0 1]
  iiwa_joint_1_AxisInvTransform : sm_lib/Frames and Transforms/Rigid Transform  TranslationMethod=Cartesian  TranslationStandardOffset=0  TranslationLengthUnit=m  TranslationStandardAxis=+Z  TranslationCartesianOffset=[0, 0, 0]  TranslationROffset=0  TranslationROffsetUnits=m  TranslationZOffset=0  TranslationZOffsetUnits=m  TranslationThetaOffset=0  TranslationThetaOffsetUnits=deg  RotationMethod=ArbitraryAxis  RotationAngleUnits=rad  RotationStandardAxis=+Z  RotationAngle=0  RotationArbitraryAxis=[1, 0, 0]  FollAlignAxisA=+X  BaseAlignAxisA=+Y  FollAlignAxisB=+Y  BaseAlignAxisB=+Z  RotationSequenceAxes=FollowerAxes  RotationSequence=XYX  RotationSequenceAngles=[0 0 0]  RotationSequenceAnglesUnits=deg  RotationMatrix=[1 0 0; 0 1 0; 0 0 1]
  iiwa_joint_2_AxisTransform : sm_lib/Frames and Transforms/Rigid Transform  TranslationMethod=Cartesian  TranslationStandardOffset=0  TranslationLengthUnit=m  TranslationStandardAxis=+Z  TranslationCartesianOffset=[0, 0, 0]  TranslationROffset=0  TranslationROffsetUnits=m  TranslationZOffset=0  TranslationZOffsetUnits=m  TranslationThetaOffset=0  TranslationThetaOffsetUnits=deg  RotationMethod=ArbitraryAxis  RotationAngleUnits=rad  RotationStandardAxis=+Z  RotationAngle=0  RotationArbitraryAxis=[1, 0, 0]  FollAlignAxisA=+X  BaseAlignAxisA=+Y  FollAlignAxisB=+Y  BaseAlignAxisB=+Z  RotationSequenceAxes=FollowerAxes  RotationSequence=XYX  RotationSequenceAngles=[0 0 0]  RotationSequenceAnglesUnits=deg  RotationMatrix=[1 0 0; 0 1 0; 0 0 1]
  iiwa_joint_2_OriginTransform : sm_lib/Frames and Transforms/Rigid Transform  TranslationMethod=Cartesian  TranslationStandardOffset=0  TranslationLengthUnit=m  TranslationStandardAxis=+Z  TranslationCartesianOffset=[0, 0, 0.19]  TranslationROffset=0  TranslationROffsetUnits=m  TranslationZOffset=0  TranslationZOffsetUnits=m  TranslationThetaOffset=0  TranslationThetaOffsetUnits=deg  RotationMethod=RotationSequence  RotationAngleUnits=deg  RotationStandardAxis=+Z  RotationAngle=0.0  RotationArbitraryAxis=[0 0 1]  FollAlignAxisA=+X  BaseAlignAxisA=+Y  FollAlignAxisB=+Y  BaseAlignAxisB=+Z  RotationSequenceAxes=BaseAxes  RotationSequence=XYZ  RotationSequenceAngles=[1.57079632679, 0, 3.14159265359]  RotationSequenceAnglesUnits=rad  RotationMatrix=[1 0 0; 0 1 0; 0 0 1]
  F : PMIOPort  Side=Left
  F1 : PMIOPort  Port=2  Side=Right
  connections:
  Inertia/RConn1 -- InertiaOriginTransform/RConn1
  InertiaOriginTransform/LConn1 -- iiwa_joint_1_AxisInvTransform/LConn1 -- iiwa_joint_2_OriginTransform/LConn1 -- VisualOriginTransform/LConn1 -- ReferenceFrame/RConn1
  Visual/RConn1 -- VisualOriginTransform/RConn1
  iiwa_joint_1_AxisInvTransform/RConn1 -- F/RConn1
  iiwa_joint_2_AxisTransform/RConn1 -- F1/RConn1
  iiwa_joint_2_AxisTransform/LConn1 -- iiwa_joint_2_OriginTransform/RConn1

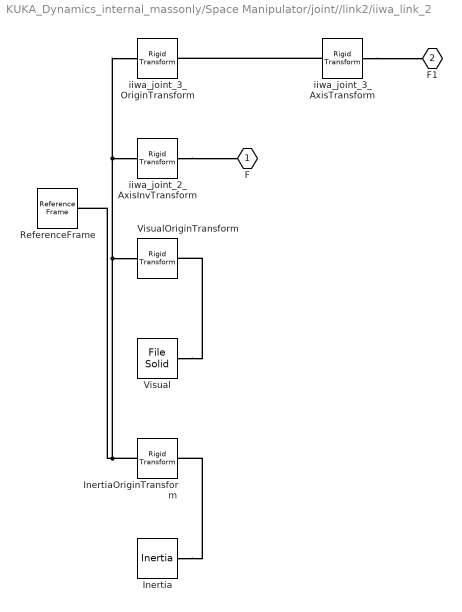
== system KUKA_Dynamics_internal_massonly/Space Manipulator/joint//link2/iiwa_link_2 ==
  Inertia : sm_lib/Body Elements/Inertia  InertiaType=Custom  Mass=3.4821  MassUnits=kg  CenterOfMass=[0, 0, 0]  CenterOfMassUnits=m  MomentsOfInertia=[0.02076, 0.02179, 0.00779]  MomentsOfInertiaUnits=kg*m^2  ProductsOfInertia=[0, -0.003626, 0]  ProductsOfInertiaUnits=kg*m^2  GraphicType=None  MarkerShape=Inertia  MarkerSize=20  GraphicVisPropType=SimpleVisualProperties  GraphicDiffuseColor=[0.5 0.5 0.5]  GraphicSpecularColor=[0.5 0.5 0.5 1.0]  GraphicAmbientColor=[0.15 0.15 0.15 1.0]  GraphicEmissiveColor=[0.0 0.0 0.0 1.0]  GraphicShininess=75  GraphicOpacity=1.0
  InertiaOriginTransform : sm_lib/Frames and Transforms/Rigid Transform  TranslationMethod=Cartesian  TranslationStandardOffset=0  TranslationLengthUnit=m  TranslationStandardAxis=+Z  TranslationCartesianOffset=[0.0003, 0.059, 0.042]  TranslationROffset=0  TranslationROffsetUnits=m  TranslationZOffset=0  TranslationZOffsetUnits=m  TranslationThetaOffset=0  TranslationThetaOffsetUnits=deg  RotationMethod=RotationSequence  RotationAngleUnits=deg  RotationStandardAxis=+Z  RotationAngle=0.0  RotationArbitraryAxis=[0 0 1]  FollAlignAxisA=+X  BaseAlignAxisA=+Y  FollAlignAxisB=+Y  BaseAlignAxisB=+Z  RotationSequenceAxes=BaseAxes  RotationSequence=XYZ  RotationSequenceAngles=[0, 0, 0]  RotationSequenceAnglesUnits=rad  RotationMatrix=[1 0 0; 0 1 0; 0 0 1]
  ReferenceFrame : sm_lib/Frames and Transforms/Reference Frame
  Visual : sm_lib/Body Elements/File Solid  ExtGeomFileName=iiwa_description/meshes/iiwa7/visual/link_2.stl  UnitType=Custom  ExtGeomFileUnits=m  StepReaderType=HEX  ExportConvexHullGeometry=off  InertiaType=Custom  Mass=0  MassUnits=kg  CenterOfMass=[0, 0, 0]  CenterOfMassUnits=m  MomentsOfInertia=[0, 0, 0]  MomentsOfInertiaUnits=kg*m^2  ProductsOfInertia=[0, 0, 0]  ProductsOfInertiaUnits=kg*m^2  BasedOnType=DensityFromFile  Density=1000  DensityUnits=kg/m^3  DoExposeReferenceFrame=on  SerializedFrames=<Frames/>  GraphicType=FromGeometry  MarkerShape=Sphere  MarkerSize=10  GraphicVisPropType=SimpleVisualProperties  GraphicDiffuseColor=[1, 0.423529411765, 0.0392156862745]  GraphicSpecularColor=[0.5 0.5 0.5 1.0]  GraphicAmbientColor=[0.15 0.15 0.15 1.0]  GraphicEmissiveColor=[0.0 0.0 0.0 1.0]  GraphicShininess=75  GraphicOpacity=1
  VisualOriginTransform : sm_lib/Frames and Transforms/Rigid Transform  TranslationMethod=Cartesian  TranslationStandardOffset=0  TranslationLengthUnit=m  TranslationStandardAxis=+Z  TranslationCartesianOffset=[0, 0, 0]  TranslationROffset=0  TranslationROffsetUnits=m  TranslationZOffset=0  TranslationZOffsetUnits=m  TranslationThetaOffset=0  TranslationThetaOffsetUnits=deg  RotationMethod=RotationSequence  RotationAngleUnits=deg  RotationStandardAxis=+Z  RotationAngle=0.0  RotationArbitraryAxis=[0 0 1]  FollAlignAxisA=+X  BaseAlignAxisA=+Y  FollAlignAxisB=+Y  BaseAlignAxisB=+Z  RotationSequenceAxes=BaseAxes  RotationSequence=XYZ  RotationSequenceAngles=[0, 0, 0]  RotationSequenceAnglesUnits=rad  RotationMatrix=[1 0 0; 0 1 0; 0 0 1]
  iiwa_joint_2_AxisInvTransform : sm_lib/Frames and Transforms/Rigid Transform  TranslationMethod=Cartesian  TranslationStandardOffset=0  TranslationLengthUnit=m  TranslationStandardAxis=+Z  TranslationCartesianOffset=[0, 0, 0]  TranslationROffset=0  TranslationROffsetUnits=m  TranslationZOffset=0  TranslationZOffsetUnits=m  TranslationThetaOffset=0  TranslationThetaOffsetUnits=deg  RotationMethod=ArbitraryAxis  RotationAngleUnits=rad  RotationStandardAxis=+Z  RotationAngle=0  RotationArbitraryAxis=[1, 0, 0]  FollAlignAxisA=+X  BaseAlignAxisA=+Y  FollAlignAxisB=+Y  BaseAlignAxisB=+Z  RotationSequenceAxes=FollowerAxes  RotationSequence=XYX  RotationSequenceAngles=[0 0 0]  RotationSequenceAnglesUnits=deg  RotationMatrix=[1 0 0; 0 1 0; 0 0 1]
  iiwa_joint_3_AxisTransform : sm_lib/Frames and Transforms/Rigid Transform  TranslationMethod=Cartesian  TranslationStandardOffset=0  TranslationLengthUnit=m  TranslationStandardAxis=+Z  TranslationCartesianOffset=[0, 0, 0]  TranslationROffset=0  TranslationROffsetUnits=m  TranslationZOffset=0  TranslationZOffsetUnits=m  TranslationThetaOffset=0  TranslationThetaOffsetUnits=deg  RotationMethod=ArbitraryAxis  RotationAngleUnits=rad  RotationStandardAxis=+Z  RotationAngle=0  RotationArbitraryAxis=[1, 0, 0]  FollAlignAxisA=+X  BaseAlignAxisA=+Y  FollAlignAxisB=+Y  BaseAlignAxisB=+Z  RotationSequenceAxes=FollowerAxes  RotationSequence=XYX  RotationSequenceAngles=[0 0 0]  RotationSequenceAnglesUnits=deg  RotationMatrix=[1 0 0; 0 1 0; 0 0 1]
  iiwa_joint_3_OriginTransform : sm_lib/Frames and Transforms/Rigid Transform  TranslationMethod=Cartesian  TranslationStandardOffset=0  TranslationLengthUnit=m  TranslationStandardAxis=+Z  TranslationCartesianOffset=[0, 0.21, 0]  TranslationROffset=0  TranslationROffsetUnits=m  TranslationZOffset=0  TranslationZOffsetUnits=m  TranslationThetaOffset=0  TranslationThetaOffsetUnits=deg  RotationMethod=RotationSequence  RotationAngleUnits=deg  RotationStandardAxis=+Z  RotationAngle=0.0  RotationArbitraryAxis=[0 0 1]  FollAlignAxisA=+X  BaseAlignAxisA=+Y  FollAlignAxisB=+Y  BaseAlignAxisB=+Z  RotationSequenceAxes=BaseAxes  RotationSequence=XYZ  RotationSequenceAngles=[1.57079632679, 0, 3.14159265359]  RotationSequenceAnglesUnits=rad  RotationMatrix=[1 0 0; 0 1 0; 0 0 1]
  F : PMIOPort  Side=Left
  F1 : PMIOPort  Port=2  Side=Right
  connections:
  Inertia/RConn1 -- InertiaOriginTransform/RConn1
  InertiaOriginTransform/LConn1 -- ReferenceFrame/RConn1 -- iiwa_joint_2_AxisInvTransform/LConn1 -- iiwa_joint_3_OriginTransform/LConn1 -- VisualOriginTransform/LConn1
  Visual/RConn1 -- VisualOriginTransform/RConn1
  iiwa_joint_2_AxisInvTransform/RConn1 -- F/RConn1
  iiwa_joint_3_AxisTransform/RConn1 -- F1/RConn1
  iiwa_joint_3_AxisTransform/LConn1 -- iiwa_joint_3_OriginTransform/RConn1
